simulink model "modelo_nao_linear"  (R2026a)
settings: Solver=VariableStepAuto  StopTime=10  MaxStep=1e-3
values from neighbouring files (symbols this model uses):
  A = 1.19    [vehicle_parameters.m]
  Bx = 16.5    [simu2.m]    (also in simu3.m; vehicle_parameters.m)
  By = 18.4    [vehicle_parameters.m]
  Cd = 1.3    [vehicle_parameters.m]
  Cl = -3.5    [vehicle_parameters.m]
  CoPF = 0.68    [vehicle_parameters.m]
  CoPR = 0.86    [vehicle_parameters.m]
  Cx = 1.4    [simu2.m]    (also in simu3.m; vehicle_parameters.m)
  Cy = 1.45    [vehicle_parameters.m]
  Dx = 1.4    [simu2.m]    (also in simu3.m; vehicle_parameters.m)
  Dy = 1.4    [vehicle_parameters.m]
  Ex = -1    [simu2.m]    (also in simu3.m; vehicle_parameters.m)
  Ey = -0.3    [vehicle_parameters.m]
  G = 9.81    [vehicle_parameters.m]
  h = 0.27    [vehicle_parameters.m]
  Iz = 120    [vehicle_parameters.m]
  Jf = 0.1381    [vehicle_parameters.m]
  Jr = 0.1376    [vehicle_parameters.m]
  Lf = 0.72    [vehicle_parameters.m]
  Lr = 0.82    [vehicle_parameters.m]
  m = 285    [vehicle_parameters.m]
  R = 0.2    [vehicle_parameters.m]
  rho = 1.225    [vehicle_parameters.m]
  Wb = 1.54    [vehicle_parameters.m]
settings Model: Creator=eduar  LastModifiedBy=eduar

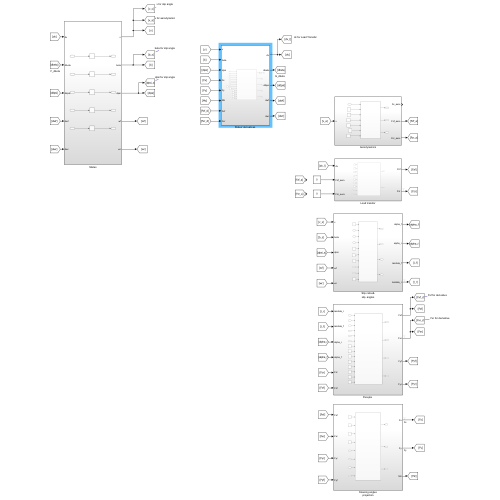
[thumbnail: Simulink's stored preview of the top-level diagram]
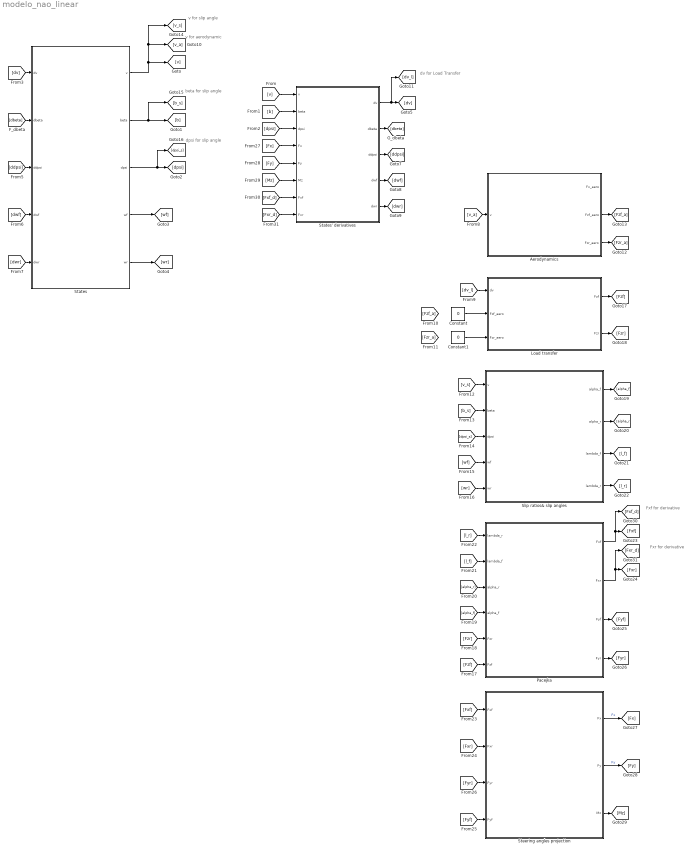
== system modelo_nao_linear ==
  note: Fxr for derivative
  note: dpsi for slip angle
  note: beta for slip angle
  note: v for slip angle
  note: dv for Load Transfer
  note: v for aerodynamic
  note: Fxf for derivative
  Aerodynamics : Subsystem
  Constant : Constant  Value=0
  Constant1 : Constant  Value=0
  Load transfer : Subsystem
  "Pacejka\t" : Subsystem
  Slip	ratios& slip	angles : Subsystem
  States : Subsystem
  "States' derivatives " : Subsystem
  Steering	angles projection : Subsystem
  wires:
  States/1(v) -> [v_a], [v_s], [v]
  States/3(dpsi) -> [dpsi_s], [dpsi]
  States/2(beta) -> [b_s], [b]
  States/4(wf) -> [wf]
  States/5(wr) -> [wr]
  [v] -> "States' derivatives "/1(v)
  [b] -> "States' derivatives "/2(beta)
  [dpsi] -> "States' derivatives "/3(dpsi)
  "States' derivatives "/1(dv) -> [dv_l], [dv]
  [dv] -> States/1(dv)
  "States' derivatives "/2(dbeta) -> [dbeta]
  [dbeta] -> States/2(dbeta)
  [ddpsi] -> States/3(ddpsi)
  [dwf] -> States/4(dwf)
  [dwr] -> States/5(dwr)
  "States' derivatives "/5(dwr) -> [dwr]
  "States' derivatives "/4(dwf) -> [dwf]
  "States' derivatives "/3(ddpsi) -> [ddpsi]
  [v_a] -> Aerodynamics/1(v)
  [dv_l] -> Load transfer/1(dv)
  Aerodynamics/2(Fzf_aero) -> [Fzf_a]
  Aerodynamics/3(Fzr_aero) -> [Fzr_a]
  [v_s] -> Slip	ratios& slip	angles/1(v)
  [b_s] -> Slip	ratios& slip	angles/2(beta)
  [dpsi_s] -> Slip	ratios& slip	angles/3(dpsi)
  [wf] -> Slip	ratios& slip	angles/4(wf)
  [wr] -> Slip	ratios& slip	angles/5(wr)
  Load transfer/1(Fzf) -> [Fzf]
  Load transfer/2(Fzr) -> [Fzr]
  [Fzf] -> "Pacejka\t"/6(Fzf)
  Slip	ratios& slip	angles/1(alpha_f) -> [alpha_f]
  Slip	ratios& slip	angles/2(alpha_r) -> [alpha_r]
  Slip	ratios& slip	angles/3(lambda_f) -> [l_f]
  Slip	ratios& slip	angles/4(lambda_r) -> [l_r]
  [l_r] -> "Pacejka\t"/1(lambda_r)
  [l_f] -> "Pacejka\t"/2(lambda_f)
  [alpha_r] -> "Pacejka\t"/3(alpha_r)
  [alpha_f] -> "Pacejka\t"/4(alpha_f)
  "Pacejka\t"/1(Fxf) -> [Fxf_d], [Fxf]
  "Pacejka\t"/4(Fyr) -> [Fyr]
  "Pacejka\t"/2(Fxr) -> [Fxr_d], [Fxr]
  "Pacejka\t"/3(Fyf) -> [Fyf]
  [Fxf] -> Steering	angles projection/1(Fxf)
  [Fxr] -> Steering	angles projection/2(Fxr)
  [Fyf] -> Steering	angles projection/4(Fyf)
  [Fyr] -> Steering	angles projection/3(Fyr)
  Steering	angles projection/1(Fx) -> [Fx]  "Fx"
  Steering	angles projection/2(Fy) -> [Fy]  "Fy"
  Steering	angles projection/3(Mz) -> [Mz]
  [Mz] -> "States' derivatives "/6(Mz)
  [Fx] -> "States' derivatives "/4(Fx)
  [Fy] -> "States' derivatives "/5(Fy)
  [Fxf_d] -> "States' derivatives "/7(Fxf)
  [Fxr_d] -> "States' derivatives "/8(Fxr)
  [Fzr] -> "Pacejka\t"/5(Fzr)
  Constant/1 -> Load transfer/2(Fzf_aero)
  Constant1/1 -> Load transfer/3(Fzr_aero)

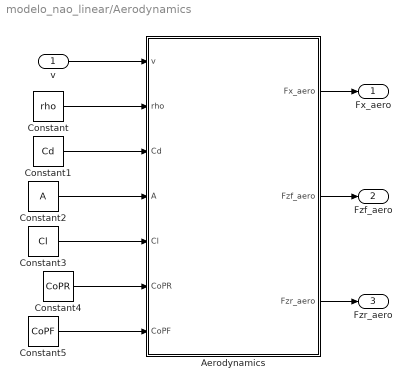
== system modelo_nao_linear/Aerodynamics ==
  v : Inport
  Aerodynamics : MATLAB Function  TreatAsAtomicUnit=on
  Constant : Constant  Value=rho
  Constant1 : Constant  Value=Cd
  Constant2 : Constant  Value=A
  Constant3 : Constant  Value=Cl
  Constant4 : Constant  Value=CoPR
  Constant5 : Constant  Value=CoPF
  Fx_aero : Outport
  Fzf_aero : Outport  Port=2
  Fzr_aero : Outport  Port=3
  wires:
  Constant/1 -> Aerodynamics/2(rho)
  Constant1/1 -> Aerodynamics/3(Cd)
  Constant2/1 -> Aerodynamics/4(A)
  Constant3/1 -> Aerodynamics/5(Cl)
  Aerodynamics/1(Fx_aero) -> Fx_aero/1
  Aerodynamics/2(Fzf_aero) -> Fzf_aero/1
  Aerodynamics/3(Fzr_aero) -> Fzr_aero/1
  v/1 -> Aerodynamics/1(v)
  Constant4/1 -> Aerodynamics/6(CoPR)
  Constant5/1 -> Aerodynamics/7(CoPF)

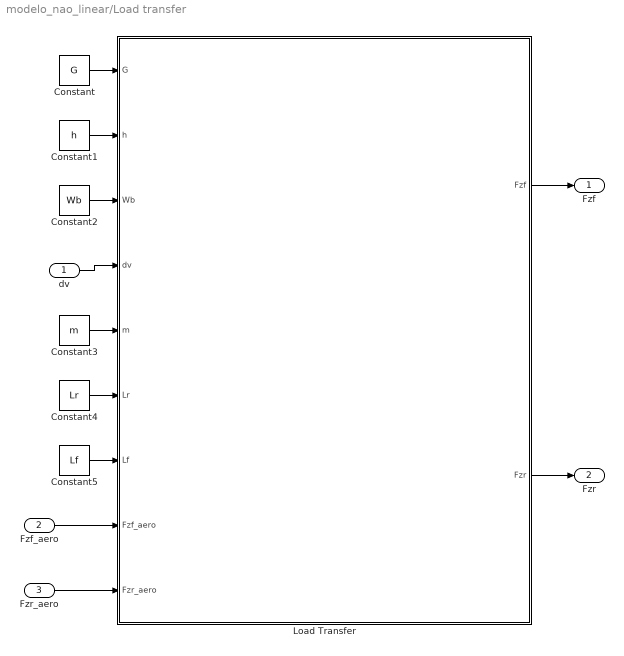
== system modelo_nao_linear/Load transfer ==
  dv : Inport
  Fzf_aero : Inport  Port=2
  Fzr_aero : Inport  Port=3
  Constant : Constant  Value=G
  Constant1 : Constant  Value=h
  Constant2 : Constant  Value=Wb
  Constant3 : Constant  Value=m
  Constant4 : Constant  Value=Lr
  Constant5 : Constant  Value=Lf
  Load Transfer : MATLAB Function  TreatAsAtomicUnit=on
  Fzf : Outport
  Fzr : Outport  Port=2
  wires:
  Constant/1 -> Load Transfer/1(G)
  Constant1/1 -> Load Transfer/2(h)
  Constant2/1 -> Load Transfer/3(Wb)
  Constant3/1 -> Load Transfer/5(m)
  Constant4/1 -> Load Transfer/6(Lr)
  Constant5/1 -> Load Transfer/7(Lf)
  Fzf_aero/1 -> Load Transfer/8(Fzf_aero)
  Fzr_aero/1 -> Load Transfer/9(Fzr_aero)
  Load Transfer/1(Fzf) -> Fzf/1
  Load Transfer/2(Fzr) -> Fzr/1
  dv/1 -> Load Transfer/4(dv)

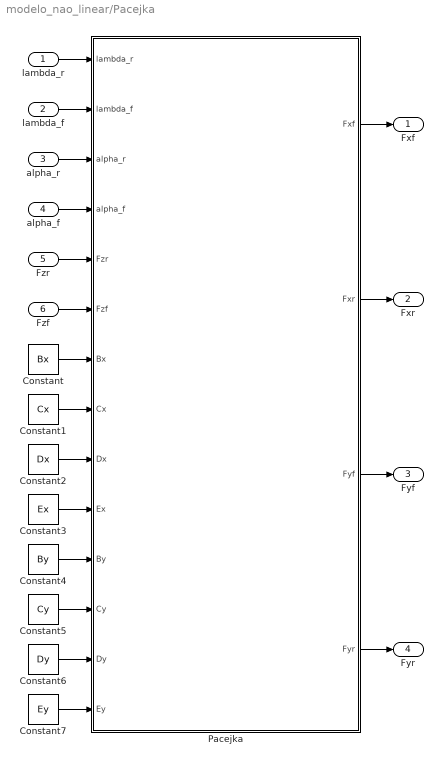
== system modelo_nao_linear/Pacejka	 ==
  lambda_r : Inport
  lambda_f : Inport  Port=2
  alpha_r : Inport  Port=3
  alpha_f : Inport  Port=4
  Fzr : Inport  Port=5
  Fzf : Inport  Port=6
  Constant : Constant  Value=Bx
  Constant1 : Constant  Value=Cx
  Constant2 : Constant  Value=Dx
  Constant3 : Constant  Value=Ex
  Constant4 : Constant  Value=By
  Constant5 : Constant  Value=Cy
  Constant6 : Constant  Value=Dy
  Constant7 : Constant  Value=Ey
  Pacejka : MATLAB Function  TreatAsAtomicUnit=on
  Fxf : Outport
  Fxr : Outport  Port=2
  Fyf : Outport  Port=3
  Fyr : Outport  Port=4
  wires:
  Constant/1 -> Pacejka/7(Bx)
  Constant1/1 -> Pacejka/8(Cx)
  Constant2/1 -> Pacejka/9(Dx)
  Constant3/1 -> Pacejka/10(Ex)
  Constant4/1 -> Pacejka/11(By)
  Constant5/1 -> Pacejka/12(Cy)
  Constant6/1 -> Pacejka/13(Dy)
  Constant7/1 -> Pacejka/14(Ey)
  lambda_r/1 -> Pacejka/1(lambda_r)
  lambda_f/1 -> Pacejka/2(lambda_f)
  alpha_r/1 -> Pacejka/3(alpha_r)
  alpha_f/1 -> Pacejka/4(alpha_f)
  Fzr/1 -> Pacejka/5(Fzr)
  Fzf/1 -> Pacejka/6(Fzf)
  Pacejka/1(Fxf) -> Fxf/1
  Pacejka/2(Fxr) -> Fxr/1
  Pacejka/3(Fyf) -> Fyf/1
  Pacejka/4(Fyr) -> Fyr/1

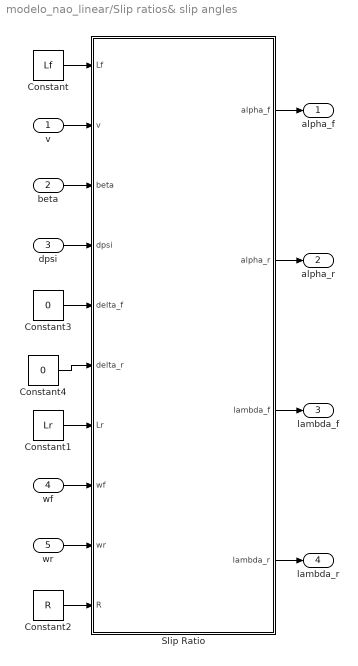
== system modelo_nao_linear/Slip	ratios& slip	angles ==
  v : Inport
  beta : Inport  Port=2
  dpsi : Inport  Port=3
  wf : Inport  Port=4
  wr : Inport  Port=5
  Constant : Constant  Value=Lf
  Constant1 : Constant  Value=Lr
  Constant2 : Constant  Value=R
  Constant3 : Constant  Value=0
  Constant4 : Constant  Value=0
  Slip Ratio : MATLAB Function  TreatAsAtomicUnit=on
  alpha_f : Outport
  alpha_r : Outport  Port=2
  lambda_f : Outport  Port=3
  lambda_r : Outport  Port=4
  wires:
  Constant2/1 -> Slip Ratio/10(R)
  Constant1/1 -> Slip Ratio/7(Lr)
  Constant/1 -> Slip Ratio/1(Lf)
  v/1 -> Slip Ratio/2(v)
  beta/1 -> Slip Ratio/3(beta)
  dpsi/1 -> Slip Ratio/4(dpsi)
  wf/1 -> Slip Ratio/8(wf)
  wr/1 -> Slip Ratio/9(wr)
  Slip Ratio/1(alpha_f) -> alpha_f/1
  Slip Ratio/2(alpha_r) -> alpha_r/1
  Slip Ratio/3(lambda_f) -> lambda_f/1
  Slip Ratio/4(lambda_r) -> lambda_r/1
  Constant4/1 -> Slip Ratio/6(delta_r)
  Constant3/1 -> Slip Ratio/5(delta_f)

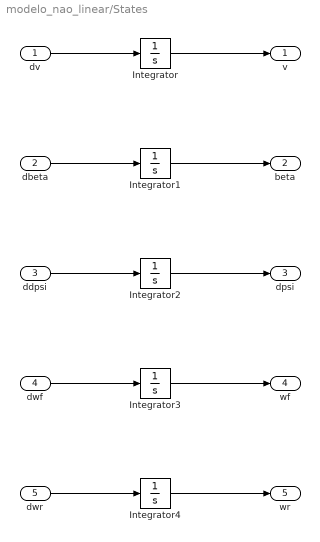
== system modelo_nao_linear/States ==
  dv : Inport  Unit=m/s
  dbeta : Inport  Port=2
  ddpsi : Inport  Port=3
  dwf : Inport  Port=4
  dwr : Inport  Port=5
  Integrator{,1..4} (5 alike) : Integrator
  v : Outport
  beta : Outport  Port=2
  dpsi : Outport  Port=3
  wf : Outport  Port=4
  wr : Outport  Port=5
  wires:
  dv/1 -> Integrator/1
  dbeta/1 -> Integrator1/1
  ddpsi/1 -> Integrator2/1
  dwf/1 -> Integrator3/1
  dwr/1 -> Integrator4/1
  Integrator/1 -> v/1
  Integrator1/1 -> beta/1
  Integrator2/1 -> dpsi/1
  Integrator3/1 -> wf/1
  Integrator4/1 -> wr/1

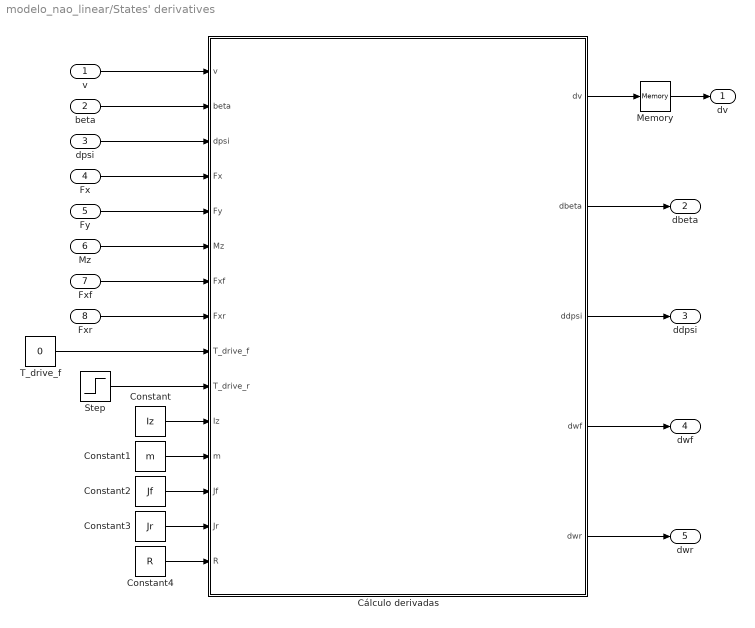
== system modelo_nao_linear/States' derivatives  ==
  v : Inport
  beta : Inport  Port=2
  dpsi : Inport  Port=3
  Fx : Inport  Port=4
  Fy : Inport  Port=5
  Mz : Inport  Port=6
  Fxf : Inport  Port=7
  Fxr : Inport  Port=8
  Constant : Constant  Value=Iz
  Constant1 : Constant  Value=m
  Constant2 : Constant  Value=Jf
  Constant3 : Constant  Value=Jr
  Constant4 : Constant  Value=R
  Cálculo derivadas : MATLAB Function  TreatAsAtomicUnit=on
  Memory : Memory
  Step : Step  FinalValue=1500  SampleTime=0
  T_drive_f : Constant  Value=0
  dv : Outport
  dbeta : Outport  Port=2
  ddpsi : Outport  Port=3
  dwf : Outport  Port=4
  dwr : Outport  Port=5
  wires:
  T_drive_f/1 -> Cálculo derivadas/9(T_drive_f)
  v/1 -> Cálculo derivadas/1(v)
  beta/1 -> Cálculo derivadas/2(beta)
  dpsi/1 -> Cálculo derivadas/3(dpsi)
  Fx/1 -> Cálculo derivadas/4(Fx)
  Fy/1 -> Cálculo derivadas/5(Fy)
  Mz/1 -> Cálculo derivadas/6(Mz)
  Fxf/1 -> Cálculo derivadas/7(Fxf)
  Fxr/1 -> Cálculo derivadas/8(Fxr)
  Cálculo derivadas/1(dv) -> Memory/1
  Cálculo derivadas/2(dbeta) -> dbeta/1
  Cálculo derivadas/3(ddpsi) -> ddpsi/1
  Cálculo derivadas/4(dwf) -> dwf/1
  Cálculo derivadas/5(dwr) -> dwr/1
  Constant/1 -> Cálculo derivadas/11(Iz)
  Constant1/1 -> Cálculo derivadas/12(m)
  Constant2/1 -> Cálculo derivadas/13(Jf)
  Constant3/1 -> Cálculo derivadas/14(Jr)
  Constant4/1 -> Cálculo derivadas/15(R)
  Step/1 -> Cálculo derivadas/10(T_drive_r)
  Memory/1 -> dv/1

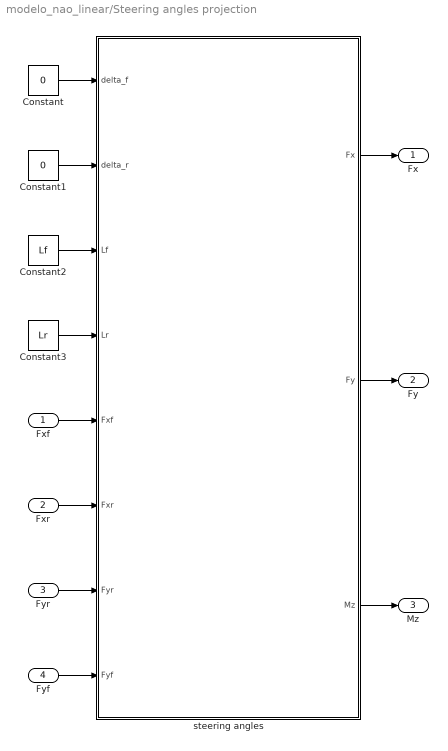
== system modelo_nao_linear/Steering	angles projection ==
  Fxf : Inport
  Fxr : Inport  Port=2
  Fyr : Inport  Port=3
  Fyf : Inport  Port=4
  Constant : Constant  Value=0
  Constant1 : Constant  Value=0
  Constant2 : Constant  Value=Lf
  Constant3 : Constant  Value=Lr
  steering angles : MATLAB Function  TreatAsAtomicUnit=on
  Fx : Outport
  Fy : Outport  Port=2
  Mz : Outport  Port=3
  wires:
  Constant/1 -> steering angles/1(delta_f)
  Constant1/1 -> steering angles/2(delta_r)
  Constant2/1 -> steering angles/3(Lf)
  Constant3/1 -> steering angles/4(Lr)
  Fxf/1 -> steering angles/5(Fxf)
  Fxr/1 -> steering angles/6(Fxr)
  Fyr/1 -> steering angles/7(Fyr)
  Fyf/1 -> steering angles/8(Fyf)
  steering angles/2(Fy) -> Fy/1
  steering angles/1(Fx) -> Fx/1
  steering angles/3(Mz) -> Mz/1

== matlab function modelo_nao_linear/Pacejka	/Pacejka ==
  data: lambda_r input; Fxf output; Fxr output; Fyf output; Fyr output; lambda_f input; alpha_r input; alpha_f input; Fzr input; Fzf input; Bx input; Cx input; Dx input; Ex input; By input; Cy input; Dy input; Ey input
function [Fxf, Fxr, Fyf, Fyr] = fcn(lambda_r, lambda_f, alpha_r, alpha_f, Fzr, Fzf, Bx, Cx, Dx, Ex, By, Cy, Dy, Ey)

Fxf = Dx * Fzf * sin(Cx * atan(Bx * lambda_f - Ex * (Bx * lambda_f - atan(Bx * lambda_f))));

Fxr = Dx * Fzr * sin(Cx * atan(Bx * lambda_r - Ex * (Bx * lambda_r - atan(Bx * lambda_r))));

Fyf = Dy * Fzf * sin(Cy * atan(By * alpha_f - Ey * (By * alpha_f - atan(By * alpha_f))));

Fyr = Dy * Fzr * sin(Cy * atan(By * alpha_r - Ey * (By * alpha_r - atan(By * alpha_r))));


end

== matlab function modelo_nao_linear/Steering	angles projection/steering angles ==
  data: delta_f input; Fx output; Fy output; Mz output; delta_r input; Lf input; Lr input; Fxf input; Fxr input; Fyr input; Fyf input
function [Fx, Fy, Mz] = fcn(delta_f, delta_r, Lf, Lr, Fxf, Fxr, Fyr, Fyf)

Fx = ( cos(delta_f) * Fxf ) - ( sin(delta_f) * Fyf ) + ( cos(delta_r) * Fxr) - ( sin(delta_r) * Fyr);

Fy = ( sin(delta_f) * Fxf ) + ( cos(delta_f) * Fyf) + ( sin(delta_r) * Fxr ) + ( cos(delta_r) * Fyr);

Mz = ( Lf*sin(delta_f) * Fxf ) + ( Lf*cos(delta_f) * Fyf ) - ( Lr*sin(delta_r) * Fxr ) - ( Lr*cos(delta_r) * Fyr );  

end

== matlab function modelo_nao_linear/Aerodynamics/Aerodynamics ==
  data: v input; Fx_aero output; Fzf_aero output; Fzr_aero output; rho input; Cd input; A input; Cl input; CoPR input; CoPF input
function [Fx_aero, Fzf_aero, Fzr_aero] = fcn(v, rho, Cd, A, Cl, CoPR, CoPF)

Fx_aero = (1/2) * rho * (v^2) * Cd * A;

Fz = (1/2) * rho * (v^2) * Cl * A;

Fzf_aero = (CoPR/(CoPR + CoPF)) * Fz;

Fzr_aero = (CoPF/(CoPR + CoPF)) * Fz;

end

== matlab function modelo_nao_linear/States' derivatives /Cálculo derivadas ==
  data: v input; dv output; beta input; dpsi input; Fx input; Fy input; Mz input; Fxf input; dbeta output; ddpsi output; Fxr input; T_drive_f input; T_drive_r input; dwf output; dwr output; Iz input; m input; Jf input; Jr input; R input
function [dv, dbeta, ddpsi, dwf, dwr] = fcn(v, beta, dpsi, Fx, Fy, Mz, Fxf, Fxr, T_drive_f, T_drive_r, Iz, m, Jf, Jr, R)
    % Parâmetros lidos diretamente do Workspace (definidos em vehicle_parameters.m):
    % m  -> Massa total do veículo
    % Iz -> Momento de inércia de guinada
    % Jf -> Momento de inércia da roda da frete
    % Jr -> Momento de inércia da roda de trás
    % R  -> Raio efetivo do pneu
    
    % Proteção contra divisão por zero na velocidade longitudinal
    if abs(v) < 1e-3
        v_safe = 1e-3;
    else
        v_safe = v;
    end
    
    % 1. Dinâmica do Corpo do Veículo (Equação 5.1 da tese)
    dv    = (cos(beta)/m) * Fx + (sin(beta)/m) * Fy;
    dbeta = (-sin(beta) / (m * v_safe)) * Fx + (cos(beta) / (m * v_safe)) * Fy - dpsi;
    ddpsi = (1 / Iz) * Mz;
    
    % 2. Dinâmica de Rotação das Rodas (Acelerações angulares)
    % Balanço de binários: Binário do motor/travão - (Força longitudinal * Raio)
    dwf = (1 / Jf) * (T_drive_f - (Fxf * R));
    dwr = (1 / Jr) * (T_drive_r - (Fxr * R));
end

== matlab function modelo_nao_linear/Load transfer/Load Transfer ==
  data: G input; Fzf output; Fzr output; h input; Wb input; dv input; m input; Lr input; Lf input; Fzf_aero input; Fzr_aero input
function [Fzf, Fzr] = fcn(G, h, Wb, dv, m, Lr, Lf, Fzf_aero, Fzr_aero)

Flt = (h/Wb) * dv * m;

Fzf_G = m * (Lr/Wb) * G;

Fzr_G = m * (Lf/Wb) * G;

Fzf = Fzf_G - Fzf_aero - Flt;

Fzr = Fzr_G - Fzr_aero + Flt;

end

== matlab function modelo_nao_linear/Slip	ratios& slip	angles/Slip Ratio ==
  data: Lf input; alpha_f output; v input; alpha_r output; lambda_f output; lambda_r output; beta input; dpsi input; delta_f input; delta_r input; Lr input; wf input; wr input; R input
function [alpha_f, alpha_r, lambda_f, lambda_r]   = fcn(Lf, v, beta, dpsi, delta_f, delta_r, Lr, wf, wr, R)

if abs(v) < 1e-3
    v_safe = 1e-3;
else
    v_safe = v;
end

% Ângulo de derrapagem da roda dianteira
alpha_f = -atan( ((v_safe * sin(beta) + Lf * dpsi) * cos(delta_f) - v_safe * cos(beta) * sin(delta_f)) / ...
    abs((v_safe * sin(beta) + Lf * dpsi) * sin(delta_f) + v_safe * cos(beta) * cos(delta_f)) );

% Ângulo de derrapagem da roda traseira
alpha_r = -atan( ((v_safe * sin(beta) - Lr * dpsi) * cos(delta_r) - v_safe * cos(beta) * sin(delta_r)) / ...
    abs((v_safe * sin(beta) - Lr * dpsi) * sin(delta_r) + v_safe * cos(beta) * cos(delta_r)) );

% Velocidade linear roda frontal
Vxf = ( v_safe * cos(beta) * cos(delta_f) ) + (v_safe * sin(beta) + Lf * dpsi) * sin(delta_f);
Vxf_safe = max(abs(Vxf), 0.1);


% Velocidade linear roda traseira
Vxr = ( v_safe * cos(beta) * cos(delta_r) ) + (v_safe * sin(beta) - Lr * dpsi) * sin(delta_r);

Vxr_safe = max(abs(Vxr), 0.1);

lambda_f = ( (wf * R) - Vxf ) / Vxf_safe ;


lambda_r =  ( (wr * R) - Vxr ) / Vxr_safe   ;

end
